simulink model "SamplingModel_4000_Abdulrahman"  (R2026a)
settings: Solver=VariableStepAuto  StopTime=20
libraries: dspxfrm3 x1, dspmlti4 x1, dspvision x1
settings Model: Creator=YazanK  LastModifiedBy=pc

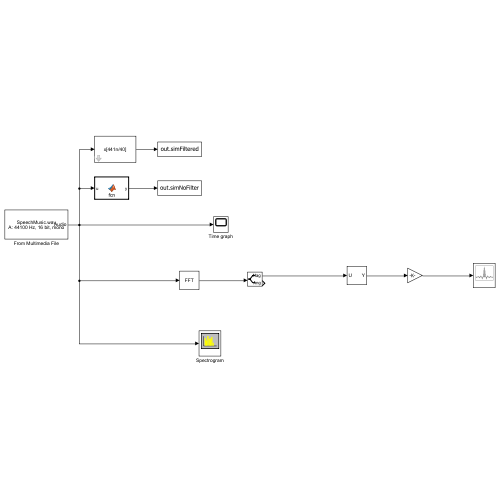
[thumbnail: Simulink's stored preview of the top-level diagram]
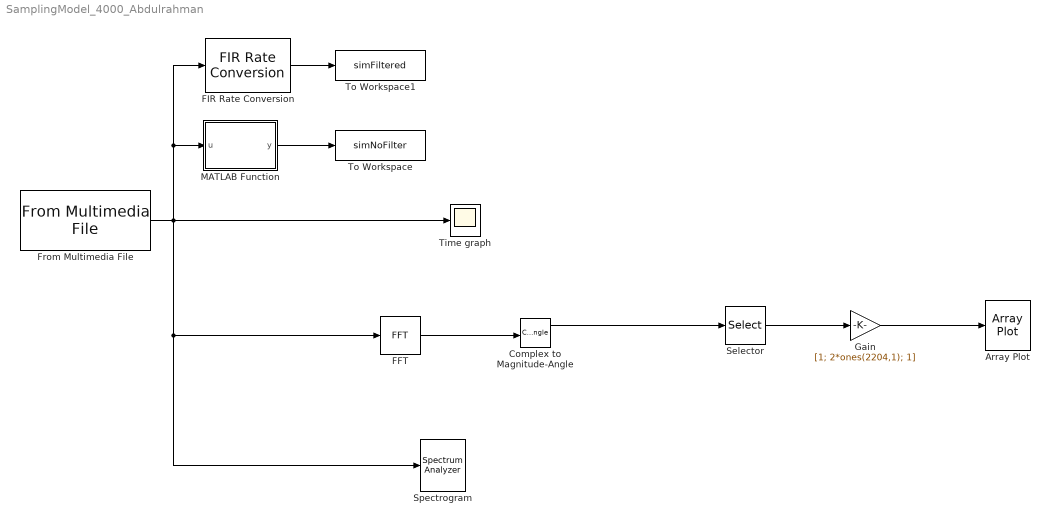
== system SamplingModel_4000_Abdulrahman ==
  Array Plot : ArrayPlot  WindowPosition=[164.000000,123.000000,808.000000,611.000000,]  ScopeFrameLocation=window  SampleIncrement=10  MaximizeAxes=Off  YLimits=[-0.0000041101 0.0000560993]
  Complex to Magnitude-Angle : ComplexToMagnitudeAngle
  FFT : dspxfrm3/FFT  FFTImplementation=Auto  CompMethod=Table lookup  TableOpt=NEW  TableOptActive=Speed  BitRevOrder=off  Normalize=on  InheritFFTLength=on  FFTLength=64  WrapInput=on  roundingMode=Ceiling  overflowMode=off  firstCoeffDataTypeStr=Inherit: Same word length as input  firstCoeffLastDataTypeStr=Inherit: Same word length as input  outputMin=[]  outputMax=[]
  FIR Rate Conversion : dspmlti4/FIR Rate Conversion  FilterSource=Dialog parameters  L=40  h=filterCoefficients4000  M=441  FilterObject=FRC  rateMode=Enforce single-rate processing  AllowArbitraryInputLength=off  roundingMode=Floor  overflowMode=off  firstCoeffDataTypeStr=Inherit: Same word length as input  firstCoeffMin=[]  firstCoeffMax=[]  firstCoeffLastDataTypeStr=Inherit: Same word length as input  outputDataTypeStr=Inherit: Same as accumulator  outputMin=[]  outputMax=[]  outputLastDataTypeStr=Inherit: Same as accumulator
  From Multimedia File : dspvision/From Multimedia File  inputFilename=Audios/SpeechMusic.wav  readRange=[1 Inf]  loop=on  numPlays=1  outputStreams=Audio only  videoDataType=single  audioDataType=double  inheritSampleTime=on  userDefinedSampleTime=1/30  noAudioOutput=off  isIntensityVideo=off  fourcc=RGB  colorVideoFormat=One multidimensional signal  outputEOF=off  dataOrg=Column-major  audioFrameSize=4410  computeAudioFrameSize=off  outSamplingMode=Sample based
      settings: LibrarySourceBlock=dspsrcs4/From Multimedia File
  Gain : Gain  Gain=[1; 2*ones(2204,1); 1]
  MATLAB Function : MATLAB Function  TreatAsAtomicUnit=on
  Selector : Selector  InputPortWidth=4410  IndexOptions=Index vector (dialog)  Indices=1:2206  OutputSizes=1
  Spectrogram : SpectrumAnalyzer  WindowPosition=[1.000000,49.000000,1536.000000,793.000000,]  ScopeFrameLocation=window  SpectrumType=Power density  ViewType=Spectrogram  Method=Welch  PlotAsTwoSidedSpectrum=off  FrequencyResolutionMethod=Window length  WindowInvariantSamplesPerUpdate=on  WindowLength=1323  FFTLengthSource=Property  FFTLength=2048  Span=22050  CenterFrequency=11025  StartFrequency=0  StopFrequency=22050  Window=Hamming  OverlapPercent=66.7  SpectrumUnits=dBW/Hz  TimeOrientation=Horizontal  TimeSpanSource=Property  TimeSpan=20  MaximizeAxes=Off  YLimits=[-120.8854793133496 7.496120686650402]  ColorLimits=[-132.38191 -41.50127]  AxesLayout=Horizontal  SelectedToolstripTab=spectrumAnalyzerToolstrip.spectrogramTab  DataDisplayPrecision=5
  Time graph : Scope
      settings: TimeUnits=Metric (based on Time Span)  ActiveDisplayYMinimum=-1.156982421875  ActiveDisplayYMaximum=1.21209716796875  YLabel=Amplitude
  To Workspace : ToWorkspace  VariableName=simNoFilter  SaveFormat=Timeseries  SampleTime=-1
  To Workspace1 : ToWorkspace  VariableName=simFiltered  SaveFormat=Timeseries  SampleTime=-1
  wires:
  From Multimedia File/1 -> FFT/1, Spectrogram/1, Time graph/1, MATLAB Function/1(u), FIR Rate Conversion/1
  FFT/1 -> Complex to Magnitude-Angle/1
  Complex to Magnitude-Angle/1 -> Selector/1
  Selector/1 -> Gain/1
  Gain/1 -> Array Plot/1
  MATLAB Function/1(y) -> To Workspace/1
  FIR Rate Conversion/1 -> To Workspace1/1

== matlab function SamplingModel_4000_Abdulrahman/MATLAB Function ==
  data: u input; y output
function y = fcn(u)
% Convert 4410 input samples to 400 samples without an AA LPF.
inputPositions = (0:4409)';
outputPositions = (0:399)' * 441 / 40;

y = interp1(inputPositions, u, outputPositions, 'linear');
end
